simulink model "PX4MultiCopterPerceptionAndControl"  (R2026b)
settings: Solver=ode3  StopTime=inf
PreLoadFcn:
  | InitVars;
undefined symbols (not defined in the file): contact, control, dragCoeffMov, ft, g, gray, m, mass, NoOfRotors, NoOfRotorsSimulation, rotorDir, rotorPositions, rotorThrustMax, rotorTimeConst, rotorTorqueMax, s, SampleTime, Sim3dSensor, Sim3dVisualisationSampleTime, windVel
libraries: aerolibconvert2 x4, sim3dlib x4, slpidlib x4, shared6dof x1, visiongeotforms x1, sharedtransform x1, uavutilslib x1
settings Model: Creator=The MathWorks, Inc.  LastModifiedBy=Hirthick
settings OptimizationCC: DefaultParameterBehavior=Inlined  DifferentSizesBufferReuse=on  EfficientTunableParamExpr=on  EnhancedBackFolding=on  MaxStackSize=64  OptimizationCustomize=off  OptimizeBlockOrder=speed  PassReuseOutputArgsAs=Individual arguments  RemoveInternalMemoryZeroInit=on  RemoveRootLevelIOMemoryZeroInit=on
settings DebuggingCC: ArithmeticOperatorsInVariantConditions=warning  MergeDetectMultiDrivingBlocksExec=none  ParameterPrecisionLossMsg=none  ParameterTunabilityLossMsg=error
settings HardwareCC: ProdHWDeviceType=ARM Compatible->ARM Cortex  ProdLargestAtomicFloat=Double  ProdLargestAtomicInteger=Long
settings ModelReferenceCC: PropagateSignalLabelsOutOfModel=off
settings SFSimCC: MATLABDynamicMemAlloc=off
settings RTWCC: Description=Embedded Coder  SystemTargetFile=ert.tlc  TemplateMakefile=ert_default_tmf  Toolchain=GNU Tools for PX4 Autopilots
settings CodeAppCC: ForceParamTrailComments=on  IgnoreCustomStorageClasses=off  InsertBlockDesc=on  OperatorAnnotations=on  SFDataObjDesc=on  SimulinkDataObjDesc=on
settings ERTTargetCC: ExtModeIntrfLevel=Level2 - Open  ExtModeMexFile=ext_xcp  ExtModeStaticAlloc=on  SupportNonFinite=off  SupportVariableSizeSignals=on
settings ConfigComp: DVDefectChecker=on  DVDetectOutOfBounds=on  DVHarnessSource=Signal Editor  DVModelReferenceHarness=on  DVTestSuiteOptimization=Auto
settings SimscapeCC: SimscapeLogType=all  SimscapeNominalValues="[{\"value\":\"1\",\"unit\":\"A\"},{\"value\":\"1\",\"unit\":\"bar\"},{\"value\":\"1\",\"unit\":\"cm^2\"},{\"value\":\"1\",\"unit\":\"cm^3/s\"},{\"value\":\"1\",\"unit\":\"kJ/kg\"},{\"value\":\"1\",\"unit\":\"kW\"},{\"value\":\"1\",\"unit\":\"l\"},{\"value\":\"1\",\"unit\":\"N\"},{\"value\":\"1\",\"unit\":\"N*m\"},{\"value\":\"1\",\"unit\":\"V\"},{\"value\":\"0.001\",\"unit\":\"Wb\"}]"  SimscapeUseEnergyAccounting=off

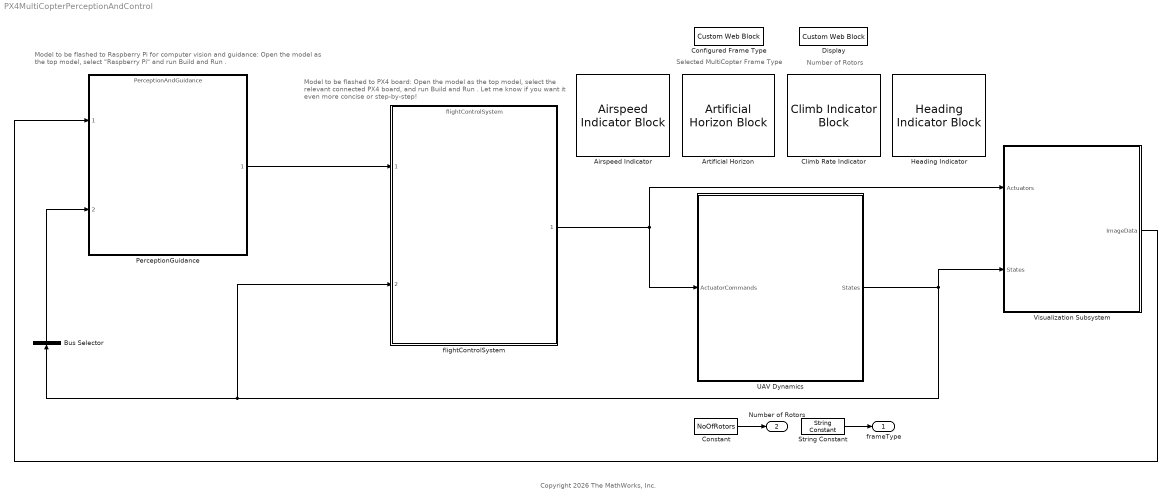
== system PX4MultiCopterPerceptionAndControl ==
  note: Selected MultiCopter Frame Type
  note: Number of Rotors
  note: Model to be flashed to Raspberry Pi for computer vision and guidance:
      | Open the model as the top model, select "Raspberry Pi" and run Build and Run .
  note: Model to be flashed to PX4 board:
      | Open the model as the top model, select the relevant connected PX4 board, and run Build and Run .
      | Let me know if you want it even more concise or step-by-step!
  note: Copyright 2026 The MathWorks, Inc.
  Airspeed Indicator : AirspeedIndicatorBlock  LabelPosition=Hide
  Artificial Horizon : ArtificialHorizonBlock  LabelPosition=Hide
  Bus Selector : BusSelector  OutputSignals=X,Y,Z,yaw  OutputAsBus=on
  Climb Rate Indicator : ClimbIndicatorBlock  LabelPosition=Hide
  "Configured Frame Type " : CustomWebBlock  LabelPosition=Hide  ShowInitialText=on  Configuration="{\"components\":[{\"name\":\"DisplayComponent\",\"settings\":{\"alignment\":\"center\",\"bold\":false,\"font\":\"Ubuntu\",\"fontColor\":[255,255,200],\"fontSize\":\"14\",\"format\":\"shortEng\",\"formatString\":\"%d\",\"gridColor\":[252,252,197],\"italic\":false,\"position\":[0,0,1,1],\"showGrid\":true,\"underline\":false}},{\"name\":\"BackgroundImageComponent\",\"settings\":{\"image\":{\"size\":[300,80],\"src\":\"data:image\\/svg+xml;base64,PHN2ZyBpZD0iZnJhbWUiIHhtbG5zPSJodHRwOi8vd3d3LnczLm9yZy8yMDAwL3N2ZyIgeG1sbnM6eGxpbms9Imh0dHA6Ly93d3cudzMub3JnLzE5OTkveGxpbmsiIHZpZXdCb3g9IjAgMCAzODAgMTAxIj48ZGVmcz48c3R5bGU+LmNscy0xe2ZpbGw6IzAwMmI0Mjt9LmNscy0ye2ZpbGw6IzQyNzA4Mjt9LmNscy0ze2ZpbGw6dXJsKCNyYWRpYWwtZ3JhZGllbnQpO308L3N0eWxlPjxyYWRpYWxHcmFkaWVudCBpZD0icmFkaWFsLWdyYWRpZW50IiBjeD0iMTkwIiBjeT0iNTAuNSIgcj0iMjY5LjIxIiBncmFkaWVudFVuaXRzPSJ1c2VyU3BhY2VPblVzZSI+PHN0b3Agb2Zmc2V0PSIwLjAxIiBzdG9wLWNvbG9yPSIjM2U0ZjU4Ii8+PHN0b3Agb2Zmc2V0PSIwLjA2IiBzdG9wLWNvbG9yPSIjNDQ1NzYxIi8+PHN0b3Agb2Zmc2V0PSIwLjE1IiBzdG9wLWNvbG9yPSIjNTU2YTc2Ii8+PHN0b3Agb2Zmc2V0PSIwLjI1IiBzdG9wLWNvbG9yPSIjNmQ4ODk1Ii8+PHN0b3Agb2Zmc2V0PSIwLjM4IiBzdG9wLWNvbG9yPSIjOGZiMmMzIi8+PHN0b3Agb2Zmc2V0PSIwLjUyIiBzdG9wLWNvbG9yPSIjYjZlNGZhIi8+PHN0b3Agb2Zmc2V0PSIxIiBzdG9wLWNvbG9yPSIjMTU0NjU3Ii8+PC9yYWRpYWxHcmFkaWVudD48L2RlZnM+PGcgaWQ9IkxheWVyXzIiIGRhdGEtbmFtZT0iTGF5ZXIgMiI+PGcgaWQ9IkxheWVyXzEtMiIgZGF0YS1uYW1lPSJMYXllciAxLTIiPjxyZWN0IGlkPSJyZWN0MTAzNiIgY2xhc3M9ImNscy0xIiB4PSIxMSIgeT0iMTEiIHdpZHRoPSIzNTgiIGhlaWdodD0iNzkiLz48cGF0aCBpZD0icGF0aDEwMzgiIGNsYXNzPSJjbHMtMiIgZD0iTTgsOFY5M0gzNzJWOFpNMzY5LDkwSDExVjExSDM2OVoiLz48cGF0aCBpZD0icGF0aDEwNDAiIGNsYXNzPSJjbHMtMyIgZD0iTTAsMFYxMDFIMzgwVjBaTTM3Miw5M0g4VjhIMzcyWiIvPjwvZz48L2c+PC9zdmc+\",\"srcOrientation\":\"Right\"},\"position\":[0,0,1,1],\"scaleMode\":\"0\"}},{\"name\":\"ForegroundImageComponent\",\"settings\":{\"angle\":0,\"image\":{\"size\":[0,0],\"src\":\"default\"},\"isForeground\":1,\"position\":[0,0,1,1],\"scaleMode\":\"0\"}}],\"derived\":{\"blockParameters\":{\"alignment\":\"center\",\"fixedAspectRatio\":\"on\",\"format\":\"shortEng\",\"formatString\":\"%d\",\"gridColor\":[252,252,197],\"showGrid\":true}},\"settings\":{\"BindingType\":\"signal\",\"aspectRatio\":1.032258064516129,\"backgroundColor\":[0,0,0,\"1\"],\"backgroundOffset\":0.14,\"backgroundOpacity\":1,\"fixedAspectRatio\":\"on\",\"showBackgroundColor\":false,\"value\":0,\"version\":\"R2026b\"},\"type\":\"Display\"}"  CustomBackgroundColor="{\"color\":[0.8509803921568627,0.8509803921568627,0.8509803921568627],\"show\":false}"
  Constant : Constant  Value=NoOfRotors  SampleTime=-1
  Display : CustomWebBlock  LabelPosition=Hide  ShowInitialText=on  Configuration="{\"components\":[{\"name\":\"DisplayComponent\",\"settings\":{\"alignment\":\"center\",\"bold\":false,\"font\":\"DSEG7 Classic\",\"fontColor\":[255,255,200],\"fontSize\":\"14\",\"format\":\"short\",\"formatString\":\"%d\",\"gridColor\":[252,252,197],\"italic\":false,\"position\":[0,0,1,1],\"showGrid\":true,\"underline\":false}},{\"name\":\"BackgroundImageComponent\",\"settings\":{\"image\":{\"size\":[300,80],\"src\":\"data:image\\/svg+xml;base64,PHN2ZyBpZD0iZnJhbWUiIHhtbG5zPSJodHRwOi8vd3d3LnczLm9yZy8yMDAwL3N2ZyIgeG1sbnM6eGxpbms9Imh0dHA6Ly93d3cudzMub3JnLzE5OTkveGxpbmsiIHZpZXdCb3g9IjAgMCAzODAgMTAxIj48ZGVmcz48c3R5bGU+LmNscy0xe2ZpbGw6IzAwMmI0Mjt9LmNscy0ye2ZpbGw6IzQyNzA4Mjt9LmNscy0ze2ZpbGw6dXJsKCNyYWRpYWwtZ3JhZGllbnQpO308L3N0eWxlPjxyYWRpYWxHcmFkaWVudCBpZD0icmFkaWFsLWdyYWRpZW50IiBjeD0iMTkwIiBjeT0iNTAuNSIgcj0iMjY5LjIxIiBncmFkaWVudFVuaXRzPSJ1c2VyU3BhY2VPblVzZSI+PHN0b3Agb2Zmc2V0PSIwLjAxIiBzdG9wLWNvbG9yPSIjM2U0ZjU4Ii8+PHN0b3Agb2Zmc2V0PSIwLjA2IiBzdG9wLWNvbG9yPSIjNDQ1NzYxIi8+PHN0b3Agb2Zmc2V0PSIwLjE1IiBzdG9wLWNvbG9yPSIjNTU2YTc2Ii8+PHN0b3Agb2Zmc2V0PSIwLjI1IiBzdG9wLWNvbG9yPSIjNmQ4ODk1Ii8+PHN0b3Agb2Zmc2V0PSIwLjM4IiBzdG9wLWNvbG9yPSIjOGZiMmMzIi8+PHN0b3Agb2Zmc2V0PSIwLjUyIiBzdG9wLWNvbG9yPSIjYjZlNGZhIi8+PHN0b3Agb2Zmc2V0PSIxIiBzdG9wLWNvbG9yPSIjMTU0NjU3Ii8+PC9yYWRpYWxHcmFkaWVudD48L2RlZnM+PGcgaWQ9IkxheWVyXzIiIGRhdGEtbmFtZT0iTGF5ZXIgMiI+PGcgaWQ9IkxheWVyXzEtMiIgZGF0YS1uYW1lPSJMYXllciAxLTIiPjxyZWN0IGlkPSJyZWN0MTAzNiIgY2xhc3M9ImNscy0xIiB4PSIxMSIgeT0iMTEiIHdpZHRoPSIzNTgiIGhlaWdodD0iNzkiLz48cGF0aCBpZD0icGF0aDEwMzgiIGNsYXNzPSJjbHMtMiIgZD0iTTgsOFY5M0gzNzJWOFpNMzY5LDkwSDExVjExSDM2OVoiLz48cGF0aCBpZD0icGF0aDEwNDAiIGNsYXNzPSJjbHMtMyIgZD0iTTAsMFYxMDFIMzgwVjBaTTM3Miw5M0g4VjhIMzcyWiIvPjwvZz48L2c+PC9zdmc+\",\"srcOrientation\":\"Right\"},\"position\":[0,0,1,1],\"scaleMode\":\"0\"}},{\"name\":\"ForegroundImageComponent\",\"settings\":{\"angle\":0,\"image\":{\"size\":[0,0],\"src\":\"default\"},\"isForeground\":1,\"position\":[0,0,1,1],\"scaleMode\":\"0\"}}],\"derived\":{\"blockParameters\":{\"alignment\":\"center\",\"fixedAspectRatio\":\"on\",\"format\":\"short\",\"formatString\":\"%d\",\"gridColor\":[252,252,197],\"showGrid\":true}},\"settings\":{\"BindingType\":\"signal\",\"aspectRatio\":1.032258064516129,\"backgroundColor\":[0,0,0,\"1\"],\"backgroundOffset\":0.14,\"backgroundOpacity\":1,\"fixedAspectRatio\":\"on\",\"showBackgroundColor\":false,\"value\":0,\"version\":\"R2026b\"},\"type\":\"Display\"}"
  Heading Indicator : HeadingIndicatorBlock  LabelPosition=Hide
  PerceptionGuidance : ModelReference  ModelNameDialog=PerceptionAndGuidance.slx  SimulationMode=Normal  ModelReferenceVersion=7.101
  String Constant : StringConstant  String=frameType
  UAV Dynamics : Subsystem
  Visualization Subsystem : Subsystem
  flightControlSystem : ModelReference  ModelNameDialog=flightControlSystem.slx  SimulationMode=Normal  ModelReferenceVersion=11.62
  frameType : Outport
  Number of Rotors : Outport  Port=2
  wires:
  flightControlSystem/1 -> Visualization Subsystem/1(Actuators), UAV Dynamics/1(ActuatorCommands)
  String Constant/1 -> frameType/1
  Constant/1 -> Number of Rotors/1
  PerceptionGuidance/1 -> flightControlSystem/1
  UAV Dynamics/1(States) -> Bus Selector/1, flightControlSystem/2, Visualization Subsystem/2(States)
  Bus Selector/1 -> PerceptionGuidance/2
  Visualization Subsystem/1(ImageData) -> PerceptionGuidance/1

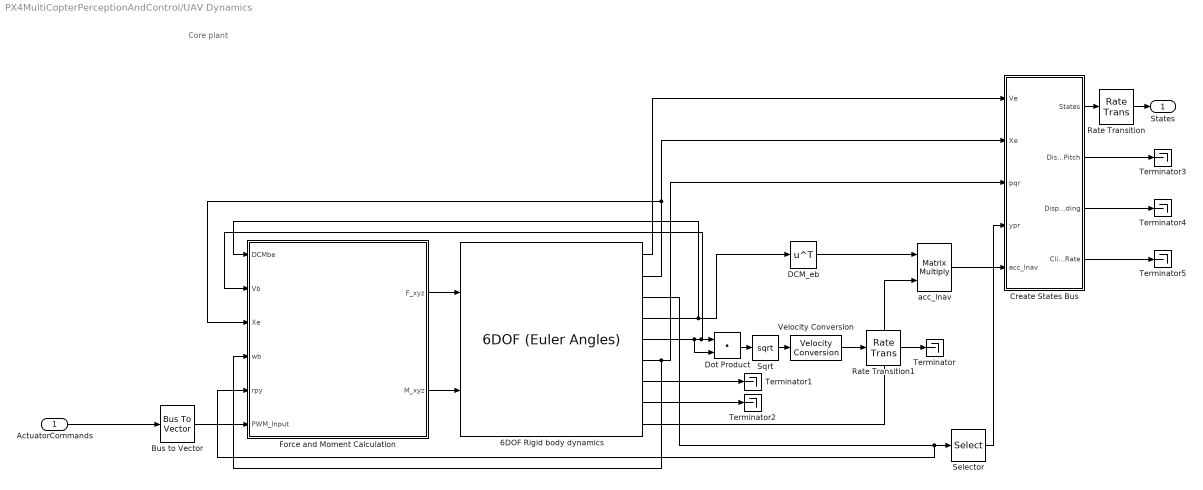
== system PX4MultiCopterPerceptionAndControl/UAV Dynamics ==
  note: Core plant
  ActuatorCommands : Inport  OutDataTypeStr=Bus: setPWMInput
  "6DOF Rigid body dynamics " : shared6dof/6DOF (Euler Angles)  units=Metric (MKS)  mtype=Fixed  rep=Euler Angles  xme_0=init.posNED  Vm_0=init.vb  eul_0=[0,0,0]  pm_0=init.angRates  mass_0=mass  mass_e=0.5  mass_f=2.0  inertia=inertia  inertia_e=eye(3)  inertia_f=2*eye(3)  k_quat=Vehicle.SixDOF.quatGain  vre_flag=on  abi_flag=on  aMode=aMode  xme_statename=''  Vm_statename=''  eul_statename=''  quat_statename=''  pm_statename=''  mass_statename=''
  Bus to Vector : BusToVector
  Create States Bus : Subsystem
  DCM_eb : Math  Operator=transpose
  Dot Product : DotProduct  OutDataTypeStr=Inherit: Inherit via internal rule
  Force and Moment Calculation : Subsystem
  Rate Transition : RateTransition  OutPortSampleTime=SampleTime
  Rate Transition1 : RateTransition
  Selector : Selector  InputPortWidth=3  IndexOptions=Index vector (dialog)  Indices=[3 2 1]  OutputSizes=1
  Sqrt : Sqrt
  Terminator{,1..5} (6 alike) : Terminator
  Velocity Conversion : aerolibconvert2/Velocity Conversion  IU=m/s  OU=kts
  acc_lnav : Product  Multiplication=Matrix(*)
  States : Outport  OutDataTypeStr=Bus: UAVStatesBus
  wires:
  "6DOF Rigid body dynamics "/3 -> Force and Moment Calculation/5(rpy), Selector/1
  "6DOF Rigid body dynamics "/8 -> Terminator2/1
  "6DOF Rigid body dynamics "/4 -> Force and Moment Calculation/1(DCMbe), DCM_eb/1
  "6DOF Rigid body dynamics "/2 -> Create States Bus/2(Xe), Force and Moment Calculation/3(Xe)
  "6DOF Rigid body dynamics "/1 -> Create States Bus/1(Ve)
  acc_lnav/1 -> Create States Bus/5(acc_lnav)
  Bus to Vector/1 -> Force and Moment Calculation/6(PWM_Input)
  "6DOF Rigid body dynamics "/7 -> Terminator1/1
  Selector/1 -> Create States Bus/4(ypr)
  Force and Moment Calculation/1(F_xyz) -> "6DOF Rigid body dynamics "/1
  DCM_eb/1 -> acc_lnav/1
  "6DOF Rigid body dynamics "/5 -> Dot Product/1, Force and Moment Calculation/2(Vb), Dot Product/2
  "6DOF Rigid body dynamics "/6 -> Force and Moment Calculation/4(wb), Create States Bus/3(pqr)
  ActuatorCommands/1 -> Bus to Vector/1
  "6DOF Rigid body dynamics "/9 -> acc_lnav/2
  Force and Moment Calculation/2(M_xyz) -> "6DOF Rigid body dynamics "/2
  Create States Bus/1(States) -> Rate Transition/1
  Rate Transition/1 -> States/1
  Create States Bus/2(DisplayRollPitch) -> Terminator3/1
  Create States Bus/3(DisplayHeading) -> Terminator4/1
  Velocity Conversion/1 -> Rate Transition1/1
  Sqrt/1 -> Velocity Conversion/1
  Dot Product/1 -> Sqrt/1
  Create States Bus/4(ClimbRate) -> Terminator5/1
  Rate Transition1/1 -> Terminator/1

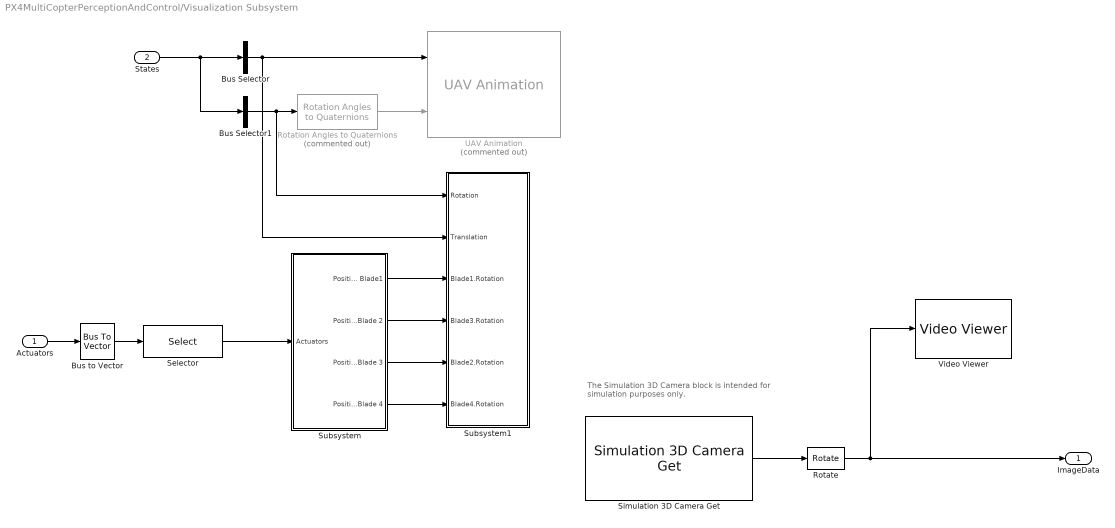
== system PX4MultiCopterPerceptionAndControl/Visualization Subsystem ==
  note: The Simulation 3D Camera block is intended for simulation purposes only.
  Actuators : Inport
  States : Inport  Port=2
  Bus Selector : BusSelector  OutputSignals=X,Y,Z  OutputAsBus=on
  Bus Selector1 : BusSelector  OutputSignals=yaw,pitch,roll  OutputAsBus=on
  Bus to Vector : BusToVector
  Rotate : visiongeotforms/Rotate  outSizeR=Expanded to fit rotated input image  src_angle=Specify via dialog  unit_angle=Degrees  angle=pi/2  maxAngle=pi  dispImage=Top-left corner  method=Table lookup  fillVal=0  interpMethod=Bilinear  roundingMode=Nearest  overflowMode=on  prodOutputMode=Binary point scaling  prodOutputWordLength=32  prodOutputFracLength=10
  Rotation Angles to Quaternions : sharedtransform/Rotation Angles to Quaternions  Commented=on  rotationOrder=ZYX  aMode=aMode
  Selector : Selector  InputPortWidth=8  IndexOptions=Index vector (dialog)  Indices=1:NoOfRotorsSimulation  OutputSizes=1
  Simulation 3D Camera Get : sim3dlib/Simulation 3D Camera Get  Priority=1  sensorTag=Sim3dSensor�  sensorId=1  sensorName=Sim3dSensor�  vehTagList={'Custom ...';'Quadcopter';'Scene Origin';'Sim3dActor1'}  vehTag=Quadcopter  CoordinateSystem=VRML  mountLoc=Origin  offsetFlag=on  tmountOffset=[0, -0.1, 0]  rmountOffset=[0, deg2rad(-90), deg2rad(90)]  HorizontalResolution=120  VerticalResolution=160  HorizontalFOV=38  SampleTime=0.2  mountPoint=[0 -0.1 0]  mountOrientation=[0 1.5707963267949 -1.5707963267949]  aMode=5  ID=1
      settings: LibrarySourceBlock=sl3dlib/Simulation 3D/Utilities/Simulation 3D Camera Get
  Subsystem : Subsystem
  Subsystem1 : Subsystem
  UAV Animation : uavutilslib/UAV Animation  Commented=on  NumUAV=1  DynamicUAVConfig=off  UAVType=Multirotor  UAVSize=1  UAVColor=[1 0 0]  UAVTrajectoryAlpha=1  AlwaysShowAnimation=on  AxisLimits=[-Inf Inf;-Inf Inf;-Inf Inf]  TrajectoryBufferSize=100000  InertialZDirection=Down  RotationFormat=Quaternion  DrawMarkers=off  SampleTime=Sim3dVisualisationSampleTime
  Video Viewer : VideoViewer  colormapValue=gray(256)  FigPos=[261 843.666666666667 419 306]
  ImageData : Outport
  wires:
  States/1 -> Bus Selector1/1, Bus Selector/1
  Subsystem/2(Position Blade 2) -> Subsystem1/4(Blade3.Rotation)
  Subsystem/4(Position Blade 4) -> Subsystem1/6(Blade4.Rotation)
  Subsystem/3(Position Blade 3) -> Subsystem1/5(Blade2.Rotation)
  Subsystem/1(Position Blade1) -> Subsystem1/3(Blade1.Rotation)
  Rotation Angles to Quaternions/1 -> UAV Animation/2
  Actuators/1 -> Bus to Vector/1
  Bus Selector1/1 -> Subsystem1/1(Rotation), Rotation Angles to Quaternions/1
  Bus Selector/1 -> Subsystem1/2(Translation), UAV Animation/1
  Selector/1 -> Subsystem/1(Actuators)
  Bus to Vector/1 -> Selector/1
  Simulation 3D Camera Get/1 -> Rotate/1
  Rotate/1 -> ImageData/1, Video Viewer/1

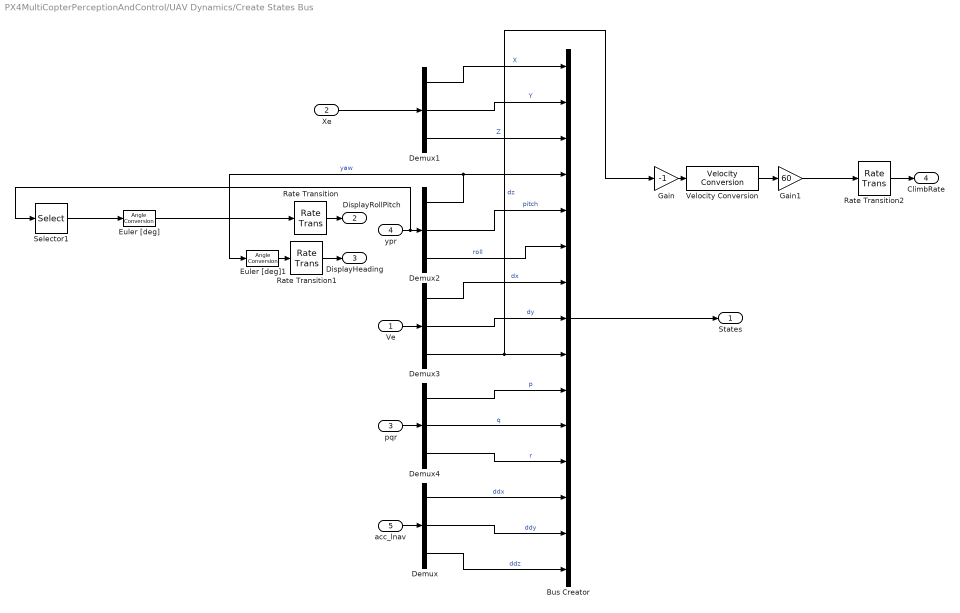
== system PX4MultiCopterPerceptionAndControl/UAV Dynamics/Create States Bus ==
  Ve : Inport
  Xe : Inport  Port=2
  pqr : Inport  Port=3
  ypr : Inport  Port=4
  acc_lnav : Inport  Port=5
  Bus Creator : BusCreator  Inputs=15
  Demux{,1..4} (5 alike) : Demux  Outputs=3
  Euler [deg] : aerolibconvert2/Angle Conversion  IU=rad  OU=deg
  Euler [deg]1 : aerolibconvert2/Angle Conversion  IU=rad  OU=deg
  Gain : Gain  Gain=-1
  Gain1 : Gain  Gain=60
  Rate Transition : RateTransition
  Rate Transition1 : RateTransition
  Rate Transition2 : RateTransition
  Selector1 : Selector  InputPortWidth=3  IndexOptions=Index vector (dialog)  Indices=[3 2]  OutputSizes=1
  Velocity Conversion : aerolibconvert2/Velocity Conversion  IU=m/s  OU=ft/s
  States : Outport
  DisplayRollPitch : Outport  Port=2
  DisplayHeading : Outport  Port=3
  ClimbRate : Outport  Port=4
  wires:
  Demux/1 -> Bus Creator/13  "ddx"
  Xe/1 -> Demux1/1
  acc_lnav/1 -> Demux/1
  Ve/1 -> Demux3/1
  pqr/1 -> Demux4/1
  Demux1/3 -> Bus Creator/3  "Z"
  Demux1/1 -> Bus Creator/1  "X"
  Demux1/2 -> Bus Creator/2  "Y"
  Demux2/1 -> Euler [deg]1/1, Bus Creator/4  "yaw"
  Demux2/2 -> Bus Creator/5  "pitch"
  Demux2/3 -> Bus Creator/6  "roll"
  Demux3/1 -> Bus Creator/7  "dx"
  Demux4/3 -> Bus Creator/12  "r"
  Demux3/2 -> Bus Creator/8  "dy"
  Demux3/3 -> Gain/1, Bus Creator/9  "dz"
  Demux4/1 -> Bus Creator/10  "p"
  Demux4/2 -> Bus Creator/11  "q"
  Demux/2 -> Bus Creator/14  "ddy"
  Demux/3 -> Bus Creator/15  "ddz"
  Bus Creator/1 -> States/1
  ypr/1 -> Selector1/1, Demux2/1
  Selector1/1 -> Euler [deg]/1
  Euler [deg]/1 -> Rate Transition/1
  Gain/1 -> Velocity Conversion/1
  Velocity Conversion/1 -> Gain1/1
  Gain1/1 -> Rate Transition2/1
  Euler [deg]1/1 -> Rate Transition1/1
  Rate Transition/1 -> DisplayRollPitch/1
  Rate Transition1/1 -> DisplayHeading/1
  Rate Transition2/1 -> ClimbRate/1

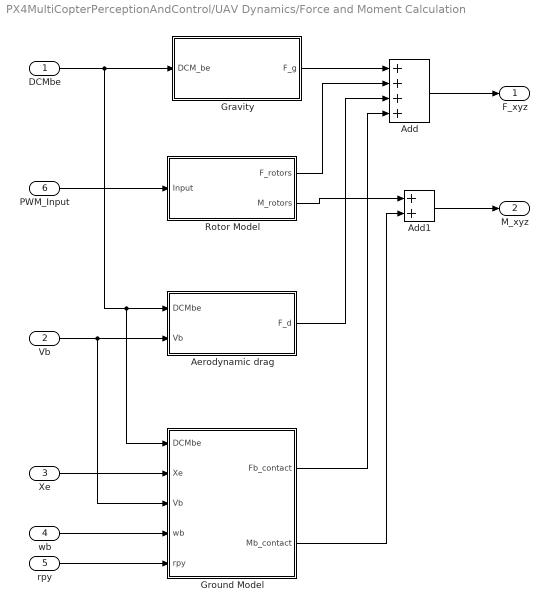
== system PX4MultiCopterPerceptionAndControl/UAV Dynamics/Force and Moment Calculation ==
  DCMbe : Inport
  Vb : Inport  Port=2
  Xe : Inport  Port=3
  wb : Inport  Port=4
  rpy : Inport  Port=5
  PWM_Input : Inport  Port=6
  Add : Sum  Inputs=++++
  Add1 : Sum
  Aerodynamic drag : Subsystem
  Gravity : Subsystem
  Ground Model : Subsystem
  Rotor Model : Subsystem
  F_xyz : Outport
  M_xyz : Outport  Port=2
  wires:
  PWM_Input/1 -> Rotor Model/1(Input)
  Gravity/1(F_g) -> Add/1
  Rotor Model/1(F_rotors) -> Add/2
  Aerodynamic drag/1(F_d) -> Add/3
  Ground Model/1(Fb_contact) -> Add/4
  Vb/1 -> Ground Model/3(Vb), Aerodynamic drag/2(Vb)
  DCMbe/1 -> Ground Model/1(DCMbe), Aerodynamic drag/1(DCMbe), Gravity/1(DCM_be)
  Xe/1 -> Ground Model/2(Xe)
  wb/1 -> Ground Model/4(wb)
  rpy/1 -> Ground Model/5(rpy)
  Rotor Model/2(M_rotors) -> Add1/1
  Ground Model/2(Mb_contact) -> Add1/2
  Add1/1 -> M_xyz/1
  Add/1 -> F_xyz/1

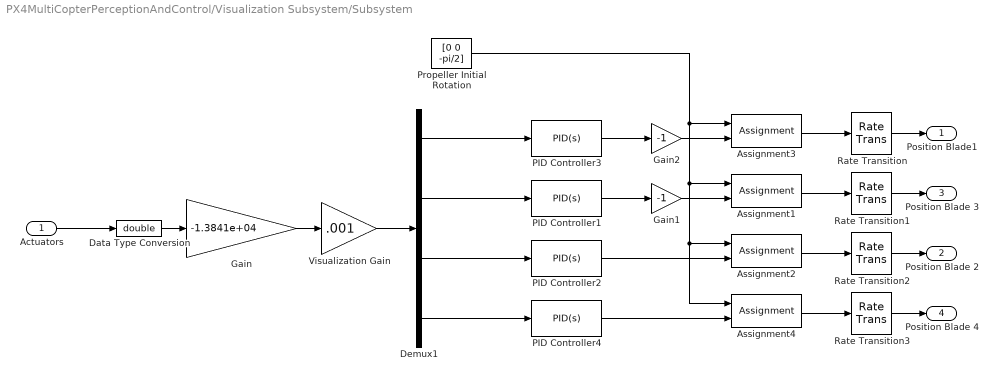
== system PX4MultiCopterPerceptionAndControl/Visualization Subsystem/Subsystem ==
  Actuators : Inport
  Assignment{1..4} (4 alike) : Assignment  DiagnosticForDimensions=Warning  IndexOptions=Index vector (dialog)  Indices=3  OutputSizes=1
  Data Type Conversion : DataTypeConversion  OutDataTypeStr=double  SaturateOnIntegerOverflow=off  RndMeth=Floor
  Demux1 : Demux
  Gain : Gain  Gain=-1.3841e+04
  Gain1 : Gain  Gain=-1
  Gain2 : Gain  Gain=-1
  PID Controller{1..4} (4 alike) : slpidlib/PID Controller  Controller=PID  Form=Parallel  TimeDomain=Continuous-time  UseExternalTs=off  SampleTime=-1  IntegratorMethod=Forward Euler  FilterMethod=Forward Euler  ControllerParametersSource=internal  P=1  I=1.5  UseKiTs=off  D=0  UseExternalDerivativeSource=off  N=100  UseFilter=on  TunerSelectOption=Transfer Function Based (PID Tuner App)  InitialConditionSource=internal  InitialConditionForIntegrator=0  InitialConditionForFilter=0  DifferentiatorICPrevScaledInput=0  ExternalReset=none  TrackingMode=off  Kt=1  LimitOutput=off  SatLimitsSource=internal  UpperSaturationLimit=inf  LowerSaturationLimit=-inf  LinearizeAsGain=on  AntiWindupMode=none  Kb=1  LimitIntegrator=off  UpperIntegratorSaturationLimit=inf  LowerIntegratorSaturationLimit=-inf  POutMin=[]  POutMax=[]  IOutMin=[]  IOutMax=[]  DOutMin=[]  DOutMax=[]  NOutMin=[]  NOutMax=[]  SumOutMin=[]  SumOutMax=[]  SaturationOutMin=[]  SaturationOutMax=[]  PParamMin=[]  PParamMax=[]  IParamMin=[]  IParamMax=[]  DParamMin=[]  DParamMax=[]  NParamMin=[]  NParamMax=[]  KbParamMin=[]  KbParamMax=[]  KtParamMin=[]  KtParamMax=[]  KbOutMin=[]  KbOutMax=[]  KtOutMin=[]  KtOutMax=[]  IntegratorOutMin=[]  IntegratorOutMax=[]  FilterOutMin=[]  FilterOutMax=[]  SumI1OutMin=[]  SumI1OutMax=[]  SumI2OutMin=[]  SumI2OutMax=[]  SumI3OutMin=[]  SumI3OutMax=[]  SumI4OutMin=[]  SumI4OutMax=[]  SumDOutMin=[]  SumDOutMax=[]  DifferentiatorOutMin=[]  DifferentiatorOutMax=[]  FilterDiffOutCoefMin=[]  FilterDiffOutCoefMax=[]  ReciprocalOutMin=[]  ReciprocalOutMax=[]  SumDenOutMin=[]  SumDenOutMax=[]  SumNumOutMin=[]  SumNumOutMax=[]  DivideOutMin=[]  DivideOutMax=[]  UdiffTsProdOutMin=[]  UdiffTsProdOutMax=[]  NTsProdOutMin=[]  NTsProdOutMax=[]  UintegralTsProdOutMin=[]  UintegralTsProdOutMax=[]  UngainTsProdOutMin=[]  UngainTsProdOutMax=[]  ClampingZeroOutDataTypeStr=Inherit: Inherit via back propagation  ClampingZeroOutMin=[]  ClampingZeroOutMax=[]  FilterDenConstantOutDataTypeStr=Inherit: Inherit via back propagation  FilterDenConstantOutMin=[]  FilterDenConstantOutMax=[]  PCopyOutDataTypeStr=Inherit: Inherit via back propagation  PCopyOutMin=[]  PCopyOutMax=[]  NCopyOutDataTypeStr=Inherit: Inherit via back propagation  NCopyOutMin=[]  NCopyOutMax=[]  IntegratorContinuousStateAttributes=''  IntegratorStateMustResolveToSignalObject=off  IntegratorRTWStateStorageClass=Auto  FilterContinuousStateAttributes=''  FilterStateMustResolveToSignalObject=off  FilterRTWStateStorageClass=Auto  ParallelPVariant=InternalParameters  IdealPVariant=Disabled  IVariant=InternalParameters  DVariant=InternalParameters  IntegratorVariant=Continuous  SatVariant=Disabled  AWVariant=Passthrough  PCopyVariant=Disabled  TRVariant=Disabled  FdbkBlocksVariant=Forward  IdealPFdbkVariant=Disabled  SatFdbkVariant=Disabled  DerivativeFilterVariant=ContFilter  NVariant=InternalParameters  NCopyVariant=Disabled  FilterICVariant=InternalICsFilter  IntegratorICVariant=InternalICs  ExternalResetVariant=Disabled  TRSumVariant=Passthrough  SumFdbkVariant=Disabled  SumVariant=Sum_PID  TsampFilterVariant=InternalTs  TsampNgainVariant=Passthrough  TsampIntegralVariant=Disabled_SignalSpec  ExternalSaturationOutDataTypeStr=Inherit: Same as second input  DerivativeSourceVariant=ErrorSignal  PreIntVariant=InternalPreInt
  Propeller Initial Rotation : Constant  Value=[0 0 -pi/2]  VectorParams1D=off  SampleTime=Sim3dVisualisationSampleTime
  Rate Transition{,1..3} (4 alike) : RateTransition
  Visualization Gain : Gain  Gain=.001
  Position Blade1 : Outport  VectorParamsAs1DForOutWhenUnconnected=off
  Position Blade 2 : Outport  Port=2  VectorParamsAs1DForOutWhenUnconnected=off
  Position Blade 3 : Outport  Port=3  VectorParamsAs1DForOutWhenUnconnected=off
  Position Blade 4 : Outport  Port=4  VectorParamsAs1DForOutWhenUnconnected=off
  wires:
  Actuators/1 -> Data Type Conversion/1
  Demux1/3 -> PID Controller2/1
  Data Type Conversion/1 -> Gain/1
  Gain/1 -> Visualization Gain/1
  Visualization Gain/1 -> Demux1/1
  Demux1/1 -> PID Controller3/1
  Demux1/2 -> PID Controller1/1
  Demux1/4 -> PID Controller4/1
  Propeller Initial Rotation/1 -> Assignment2/1, Assignment4/1, Assignment1/1, Assignment3/1
  Assignment1/1 -> Rate Transition1/1
  Assignment3/1 -> Rate Transition/1
  Assignment2/1 -> Rate Transition2/1
  Assignment4/1 -> Rate Transition3/1
  PID Controller4/1 -> Assignment4/2
  PID Controller3/1 -> Gain2/1
  PID Controller1/1 -> Gain1/1
  PID Controller2/1 -> Assignment2/2
  Gain2/1 -> Assignment3/2
  Rate Transition/1 -> Position Blade1/1
  Rate Transition1/1 -> Position Blade 3/1
  Rate Transition2/1 -> Position Blade 2/1
  Rate Transition3/1 -> Position Blade 4/1
  Gain1/1 -> Assignment1/2

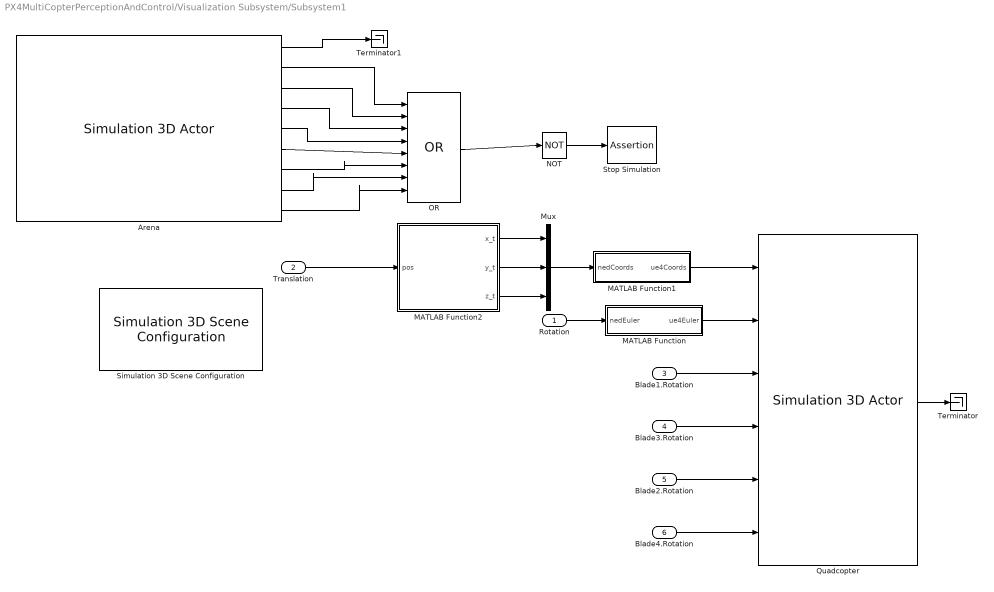
== system PX4MultiCopterPerceptionAndControl/Visualization Subsystem/Subsystem1 ==
  Rotation : Inport
  Translation : Inport  Port=2
  Blade1.Rotation : Inport  Port=3
  Blade3.Rotation : Inport  Port=4
  Blade2.Rotation : Inport  Port=5
  Blade4.Rotation : Inport  Port=6
  Arena : sim3dlib/Simulation 3D Actor  Priority=1  ActorName=Sim3dActor1  ParentName=Scene Origin  Operation=Create at setup  InitScriptText=|  SampleTime=Sim3dVisualisationSampleTime  Translation=single([0 0 0])  Rotation=single([0 0 0])  Scale=single([1 1 1])  EventsText=|  aMode=5  ActorTag=Sim3dActor1  ActorType=Sim3dActor  ID=1
      InitScriptText=|
      | % Reserved keywords:
      | % - Actor : handle to this actor object
      | % - World : handle to the world object
      | 
      | % Examples:
      | 
      | % Create a primitive geometry (optional)
      | % createShape(Actor, 'box', [1 1 1]);
      | 
      | % Initialize values (optional)
      | % Actor.Physics = true;
      | % Actor.Color = [1 0 0];
      EventsText=|
      | pillar1.BeginOverlapEvent
      | pillar2.BeginOverlapEvent
      | pillar3.BeginOverlapEvent
      | pillar4.BeginOverlapEvent
      | wall.BeginOverlapEvent   
      | wall_2.BeginOverlapEvent 
      | wall_3.BeginOverlapEvent 
      | wall_4.BeginOverlapEvent
  MATLAB Function : MATLAB Function  TreatAsAtomicUnit=on
  MATLAB Function1 : MATLAB Function  TreatAsAtomicUnit=on
  MATLAB Function2 : MATLAB Function  TreatAsAtomicUnit=on
  Mux : Mux  Inputs=3
  NOT : Logic  Operator=NOT  IconShape=distinctive  AllPortsSameDT=off  OutDataTypeStr=boolean
  OR : Logic  Operator=OR  Inputs=8  IconShape=distinctive  AllPortsSameDT=off  OutDataTypeStr=boolean
  Quadcopter : sim3dlib/Simulation 3D Actor  Priority=1  ActorName=Quadcopter  ParentName=Scene Origin  Operation=Create at setup  InitScriptText=|  SampleTime=Sim3dVisualisationSampleTime  Translation=single([0 0 0])  Rotation=single([0 0 -90])  Scale=single([1 1 1])  InputsText=|  aMode=5  ActorTag=Quadcopter  ActorType=Sim3dActor  ID=C
      InitScriptText=|
      | fileName = fullfile(fileparts(fileparts(get_param(bdroot,'FileName'))), 'support','Quadcopter.mat');
      | Actor.load(fileName);
      | Actor.Mobility=sim3d.utils.MobilityTypes.Movable;
      | World.Actors.QuadBody.Collisions = 0; % Disable Collisions
      | % propagate(World.Actors.QuadBody, 'OverlapEventEnabled',true);
      | % World.Actors.QuadBody.Translation = [-1.5 -1 0.05];
      InputsText=|
      | Quadcopter.Translation
      | Quadcopter.Rotation   
      | Prop_FR.Rotation      
      | Prop_FL.Rotation      
      | Prop_RL.Rotation      
      | Prop_RR.Rotation
  Simulation 3D Scene Configuration : sim3dlib/Simulation 3D Scene Configuration  Priority=0  EnableWindow=on  ViewerType=Default Viewer  ProjectFormat=Default Scenes  SceneDesc=US city block  ProjectName=D:\MATLAB\toolbox\shared\sim3d_projects\automotive_project_windows\UE\WindowsNoEditor\VehicleSimulation.exe  ScenePath=/Game/Maps/HwStrght  EnableOpenDRIVE=off  vehTagList={'Custom';'Quadcopter';'Scene Origin';'Sim3dActor1'}  vehTag=Quadcopter  AttachedCameraRelativeTranslation=[0 0 1]  FreeCameraDefaultInitialTranslation=[-6, 0, 2]  AttachedCameraRelativeRotation=[0 -90 0]  FreeCameraDefaultInitialRotation=[0, -15, 0]  ViewpointName=Custom  FreeCameraInitialTranslation=[2 2 6]  FreeCameraInitialRotation=[0 -90 0]  OpVisEn=off  Ts=Sim3dVisualisationSampleTime  EnableRemoteAccess=off  SimulationMode=CoSimulation  SimulateUsing=Interpreted execution  EnableAnimationRecording=off  OverrideDefaultRecording=off  AnimationRecordingFileName=sim3dAnimation.mat  AnimationRecordingInterval=[0 inf]  EnableWeather=off  SunAzimuth=90  SunAltitude=40.0  EnableGeospatialSun=off  Latitude=0  Longitude=0  Date=2023-01-01  Time=10:30:00  GeoTimeZone=-5.0  SunDaylightSaving=off  wind=1  clouds=10  EnableVolumetricClouds=off  CloudCoverage=0  CloudAltitude=6  fog=0  rain=0  RaindropsEffect=off  SnowDensity=0  EnableGeospatial=off  TilesetSource=Earth terrain  UseTrueOrigin=off  OriginHeight=200  OriginLatitude=40.744652  OriginLongitude=-73.988864  MapStyle=Aerial  AdditionalAssetIDs=[]  UseAdvancedSunSky=off  SolarTime=11  TimeZone=-5  Day=21  Month=9  Year=2022  UseDaylightSavingTime=on  DSTStartDay=10  DSTStartMonth=3  DSTEndDay=3  DSTEndMonth=11  DSTSwitchHour=2  sensorTag=MainCamera1  sensorId=1  sensorName=MainCamera1  mountLoc=Origin  offsetFlag=off  tmountOffset=[0, 0, 0]  rmountOffset=[0, 0, 0]  HorizontalResolution=1280  VerticalResolution=720  HorizontalFOV=60  mountPoint=[0 0 0]  mountOrientation=[0 0 0]  aMode=5  ID=1  GeoTrigger=Inactive  ViewNameList={'Custom'}  ViewTranslationList={'[2 2 6]'}  ViewRotationList={'[0 -90 0]'}
      settings: LibrarySourceBlock=sl3dlib/Simulation 3D/Environment/Simulation 3D Scene Configuration
  Stop Simulation : Assertion  AssertionFailFcn=error('The model has stopped as the drone hit the boundary.')
  Terminator : Terminator
  Terminator1 : Terminator
  wires:
  Arena/1 -> Terminator1/1
  MATLAB Function2/3(z_t) -> Mux/3
  Arena/2 -> OR/1
  Arena/3 -> OR/2
  Arena/4 -> OR/3
  Arena/5 -> OR/4
  OR/1 -> NOT/1
  MATLAB Function2/1(x_t) -> Mux/1
  MATLAB Function2/2(y_t) -> Mux/2
  NOT/1 -> Stop Simulation/1
  Rotation/1 -> MATLAB Function/1(nedEuler)
  MATLAB Function1/1(ue4Coords) -> Quadcopter/1
  Blade1.Rotation/1 -> Quadcopter/3
  Blade3.Rotation/1 -> Quadcopter/4
  Blade2.Rotation/1 -> Quadcopter/5
  Blade4.Rotation/1 -> Quadcopter/6
  Quadcopter/1 -> Terminator/1
  MATLAB Function/1(ue4Euler) -> Quadcopter/2
  Arena/6 -> OR/5
  Arena/7 -> OR/6
  Arena/8 -> OR/7
  Arena/9 -> OR/8
  Translation/1 -> MATLAB Function2/1(pos)
  Mux/1 -> MATLAB Function1/1(nedCoords)

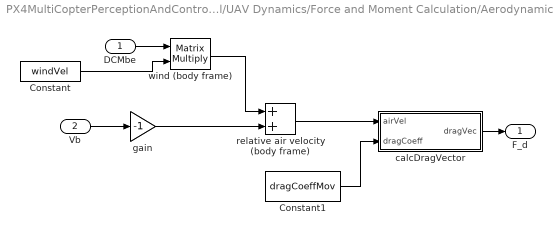
== system PX4MultiCopterPerceptionAndControl/UAV Dynamics/Force and Moment Calculation/Aerodynamic drag ==
  DCMbe : Inport
  Vb : Inport  Port=2
  Constant : Constant  Value=windVel
  Constant1 : Constant  Value=dragCoeffMov  SampleTime=-1
  calcDragVector : MATLAB Function  TreatAsAtomicUnit=on
  gain : Gain  Gain=-1
  relative air velocity (body frame) : Sum
  wind (body frame) : Product  Multiplication=Matrix(*)
  F_d : Outport
  wires:
  Vb/1 -> gain/1
  calcDragVector/1(dragVec) -> F_d/1
  relative air velocity (body frame)/1 -> calcDragVector/1(airVel)
  gain/1 -> relative air velocity (body frame)/2
  Constant1/1 -> calcDragVector/2(dragCoeff)
  DCMbe/1 -> wind (body frame)/1
  Constant/1 -> wind (body frame)/2
  wind (body frame)/1 -> relative air velocity (body frame)/1

== system PX4MultiCopterPerceptionAndControl/UAV Dynamics/Force and Moment Calculation/Gravity ==
  DCM_be : Inport
  Constant : Constant  Value=[0 0 g]'
  Gain : Gain  Gain=mass
  Matrix Multiply : Product  Multiplication=Matrix(*)
  F_g : Outport
  wires:
  Matrix Multiply/1 -> Gain/1
  Constant/1 -> Matrix Multiply/2
  DCM_be/1 -> Matrix Multiply/1
  Gain/1 -> F_g/1

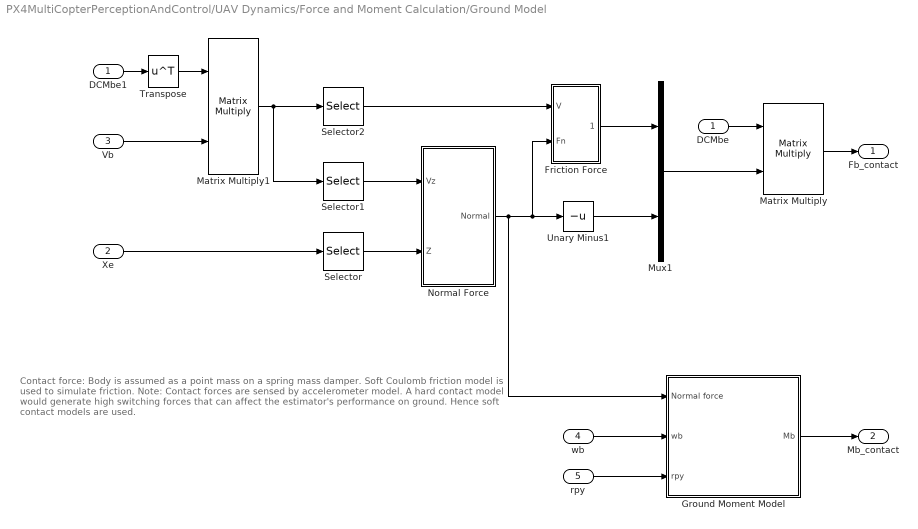
== system PX4MultiCopterPerceptionAndControl/UAV Dynamics/Force and Moment Calculation/Ground Model ==
  note: Contact force:
      | Body is assumed as a point mass on a spring mass damper. Soft Coulomb friction model is used to simulate friction.
      |
      | Note:
      | Contact forces are sensed by accelerometer model. A hard contact model would generate high switching forces that can affect the estimator's performance on ground. Hence soft contact models are used.
  DCMbe : Inport
  Xe : Inport  Port=2
  Vb : Inport  Port=3
  wb : Inport  Port=4
  rpy : Inport  Port=5
  DCMbe1 : InportShadow
  Friction Force : Subsystem
  Ground Moment Model : Subsystem
  Matrix Multiply : Product  Multiplication=Matrix(*)
  Matrix Multiply1 : Product  Multiplication=Matrix(*)
  Mux1 : Mux  Inputs=2
  Normal Force : Subsystem
  Selector : Selector  InputPortWidth=3  IndexOptions=Index vector (dialog)  Indices=[3]  OutputSizes=1
  Selector1 : Selector  InputPortWidth=3  IndexOptions=Index vector (dialog)  Indices=[3]  OutputSizes=1
  Selector2 : Selector  InputPortWidth=3  IndexOptions=Index vector (dialog)  Indices=[1,2]  OutputSizes=1
  Transpose : Math  Operator=transpose
  Unary Minus1 : UnaryMinus
  Fb_contact : Outport
  Mb_contact : Outport  Port=2
  wires:
  Xe/1 -> Selector/1
  Selector1/1 -> Normal Force/1(Vz)
  Selector/1 -> Normal Force/2(Z)
  DCMbe/1 -> Matrix Multiply/1
  Matrix Multiply/1 -> Fb_contact/1
  Normal Force/1(Normal) -> Ground Moment Model/1(Normal force), Unary Minus1/1, Friction Force/2(Fn)
  Mux1/1 -> Matrix Multiply/2
  Unary Minus1/1 -> Mux1/2
  Selector2/1 -> Friction Force/1(V)
  Friction Force/1(Friction) -> Mux1/1
  DCMbe1/1 -> Transpose/1
  Transpose/1 -> Matrix Multiply1/1
  Vb/1 -> Matrix Multiply1/2
  Matrix Multiply1/1 -> Selector1/1, Selector2/1
  Ground Moment Model/1(Mb) -> Mb_contact/1
  wb/1 -> Ground Moment Model/2(wb)
  rpy/1 -> Ground Moment Model/3(rpy)

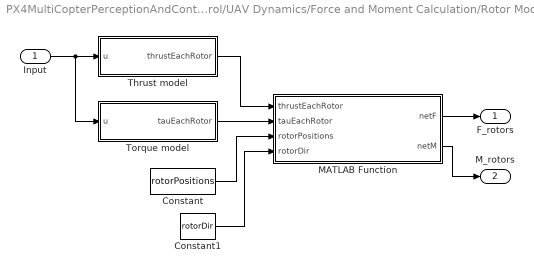
== system PX4MultiCopterPerceptionAndControl/UAV Dynamics/Force and Moment Calculation/Rotor Model ==
  Input : Inport
  Constant : Constant  Value=rotorPositions  SampleTime=-1
  Constant1 : Constant  Value=rotorDir  SampleTime=-1
  MATLAB Function : MATLAB Function  TreatAsAtomicUnit=on
  Thrust model : Subsystem
  Torque model : Subsystem
  F_rotors : Outport
  M_rotors : Outport  Port=2
  wires:
  MATLAB Function/1(netF) -> F_rotors/1
  Constant1/1 -> MATLAB Function/4(rotorDir)
  Constant/1 -> MATLAB Function/3(rotorPositions)
  Input/1 -> Thrust model/1(u), Torque model/1(u)
  Thrust model/1(thrustEachRotor) -> MATLAB Function/1(thrustEachRotor)
  Torque model/1(tauEachRotor) -> MATLAB Function/2(tauEachRotor)
  MATLAB Function/2(netM) -> M_rotors/1

== system PX4MultiCopterPerceptionAndControl/UAV Dynamics/Force and Moment Calculation/Ground Model/Friction Force ==
  V : Inport
  Fn : Inport  Port=2
  Product : Product
  Saturation : Saturate  UpperLimit=contact.translation.maxFriction  LowerLimit=-contact.translation.maxFriction
  Soft Coulomb Friction : Subsystem
  Unary Minus : UnaryMinus
  Friction : Outport
  wires:
  Fn/1 -> Product/2
  Soft Coulomb Friction/1(Out1) -> Product/1
  Product/1 -> Unary Minus/1
  V/1 -> Soft Coulomb Friction/1(In1)
  Unary Minus/1 -> Saturation/1
  Saturation/1 -> Friction/1

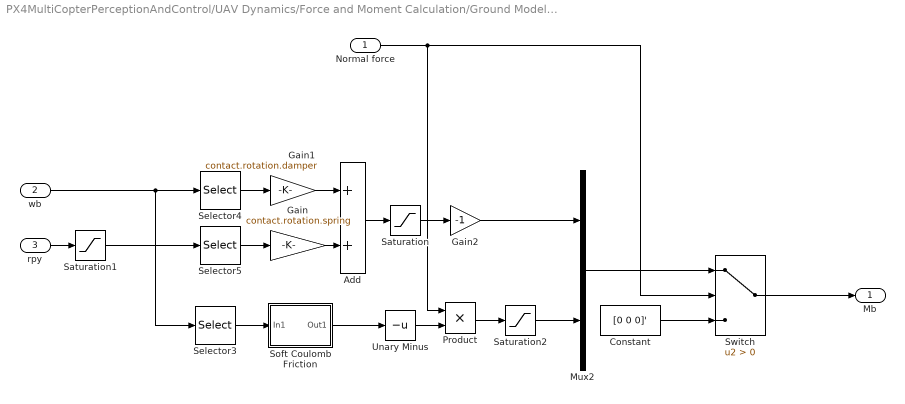
== system PX4MultiCopterPerceptionAndControl/UAV Dynamics/Force and Moment Calculation/Ground Model/Ground Moment Model ==
  Normal force : Inport
  wb : Inport  Port=2
  rpy : Inport  Port=3
  Add : Sum
  Constant : Constant  Value=[0 0 0]'
  Gain : Gain  Gain=contact.rotation.spring
  Gain1 : Gain  Gain=contact.rotation.damper
  Gain2 : Gain  Gain=-1
  Mux2 : Mux  Inputs=2
  Product : Product
  Saturation : Saturate  UpperLimit=control.rotation.maxMoment  LowerLimit=-control.rotation.maxMoment
  Saturation1 : Saturate  UpperLimit=20*pi/180  LowerLimit=-20*pi/180
  Saturation2 : Saturate  UpperLimit=control.rotation.maxMoment  LowerLimit=-control.rotation.maxMoment
  Selector3 : Selector  InputPortWidth=3  IndexOptions=Index vector (dialog)  Indices=[3]  OutputSizes=1
  Selector4 : Selector  InputPortWidth=3  IndexOptions=Index vector (dialog)  Indices=[1, 2]  OutputSizes=1
  Selector5 : Selector  InputPortWidth=3  IndexOptions=Index vector (dialog)  Indices=[1, 2]  OutputSizes=1
  Soft Coulomb Friction : Subsystem
  Switch : Switch  Criteria=u2 > Threshold  SaturateOnIntegerOverflow=off  InputSameDT=off
  Unary Minus : UnaryMinus
  Mb : Outport
  wires:
  Gain2/1 -> Mux2/1
  Add/1 -> Saturation/1
  Gain/1 -> Add/2
  Saturation/1 -> Gain2/1
  Selector4/1 -> Gain1/1
  Gain1/1 -> Add/1
  Constant/1 -> Switch/3
  Selector5/1 -> Gain/1
  Switch/1 -> Mb/1
  Mux2/1 -> Switch/1
  Normal force/1 -> Product/1, Switch/2
  rpy/1 -> Saturation1/1
  Saturation1/1 -> Selector5/1
  wb/1 -> Selector4/1, Selector3/1
  Selector3/1 -> Soft Coulomb Friction/1(In1)
  Soft Coulomb Friction/1(Out1) -> Unary Minus/1
  Unary Minus/1 -> Product/2
  Product/1 -> Saturation2/1
  Saturation2/1 -> Mux2/2

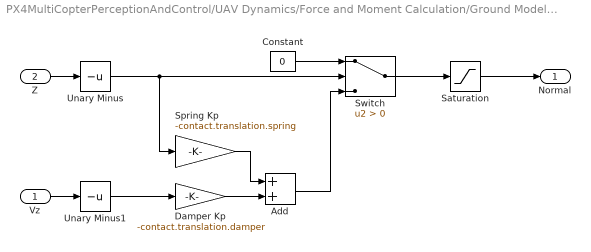
== system PX4MultiCopterPerceptionAndControl/UAV Dynamics/Force and Moment Calculation/Ground Model/Normal Force ==
  Vz : Inport
  Z : Inport  Port=2
  Add : Sum
  Constant : Constant  Value=0
  Damper Kp : Gain  Gain=-contact.translation.damper
  Saturation : Saturate  UpperLimit=contact.translation.maxNormal  LowerLimit=0
  Spring Kp : Gain  Gain=-contact.translation.spring
  Switch : Switch  Criteria=u2 > Threshold  SaturateOnIntegerOverflow=off  InputSameDT=off
  Unary Minus : UnaryMinus
  Unary Minus1 : UnaryMinus
  Normal : Outport
  wires:
  Constant/1 -> Switch/1
  Z/1 -> Unary Minus/1
  Switch/1 -> Saturation/1
  Damper Kp/1 -> Add/2
  Add/1 -> Switch/3
  Spring Kp/1 -> Add/1
  Vz/1 -> Unary Minus1/1
  Saturation/1 -> Normal/1
  Unary Minus/1 -> Spring Kp/1, Switch/2
  Unary Minus1/1 -> Damper Kp/1

== system PX4MultiCopterPerceptionAndControl/UAV Dynamics/Force and Moment Calculation/Rotor Model/Thrust model ==
  u : Inport
  Constant : Constant  Value=rotorThrustMax  SampleTime=SampleTime
  Constant1 : Constant  Value=rotorTimeConst  SampleTime=SampleTime
  Constant2 : Constant  Value=SampleTime  SampleTime=SampleTime
  MATLAB Function : MATLAB Function  TreatAsAtomicUnit=on
  Rate Transition1 : RateTransition
  Selector : Selector  InputPortWidth=8  IndexOptions=Index vector (dialog)  Indices=1:NoOfRotors  OutputSizes=1
  thrustEachRotor : Outport
  wires:
  u/1 -> Selector/1
  Selector/1 -> MATLAB Function/1(u)
  MATLAB Function/1(y) -> Rate Transition1/1
  Constant1/1 -> MATLAB Function/4(tau)
  Constant/1 -> MATLAB Function/3(K)
  Constant2/1 -> MATLAB Function/2(Ts)
  Rate Transition1/1 -> thrustEachRotor/1

== system PX4MultiCopterPerceptionAndControl/UAV Dynamics/Force and Moment Calculation/Rotor Model/Torque model ==
  u : Inport
  Constant : Constant  Value=rotorTorqueMax  SampleTime=SampleTime
  Constant1 : Constant  Value=rotorTimeConst  SampleTime=SampleTime
  Constant2 : Constant  Value=SampleTime  SampleTime=SampleTime
  MATLAB Function : MATLAB Function  TreatAsAtomicUnit=on
  Rate Transition : RateTransition
  Selector : Selector  InputPortWidth=8  IndexOptions=Index vector (dialog)  Indices=1:NoOfRotors  OutputSizes=1
  tauEachRotor : Outport
  wires:
  Constant1/1 -> MATLAB Function/4(tau)
  u/1 -> Selector/1
  MATLAB Function/1(y) -> Rate Transition/1
  Selector/1 -> MATLAB Function/1(u)
  Constant/1 -> MATLAB Function/3(K)
  Constant2/1 -> MATLAB Function/2(Ts)
  Rate Transition/1 -> tauEachRotor/1

== system PX4MultiCopterPerceptionAndControl/UAV Dynamics/Force and Moment Calculation/Ground Model/Friction Force/Soft Coulomb Friction ==
  note: Pennestrì, E., Rossi, V., Salvini, P. et al. Review and comparison of dry friction force models. Nonlinear Dyn 83, 1785–1801 (2016). https://doi.org/10.1007/s11071-015-2485-3
  In1 : Inport
  Tanh : Trigonometry  Operator=tanh
  friction coefficient : Gain  Gain=contact.translation.friction
  vd : Gain  Gain=1/contact.translation.vd
  Out1 : Outport
  wires:
  In1/1 -> vd/1
  vd/1 -> Tanh/1
  Tanh/1 -> friction coefficient/1
  friction coefficient/1 -> Out1/1

== system PX4MultiCopterPerceptionAndControl/UAV Dynamics/Force and Moment Calculation/Ground Model/Ground Moment Model/Soft Coulomb Friction ==
  note: Pennestrì, E., Rossi, V., Salvini, P. et al. Review and comparison of dry friction force models. Nonlinear Dyn 83, 1785–1801 (2016). https://doi.org/10.1007/s11071-015-2485-3
  In1 : Inport
  Tanh : Trigonometry  Operator=tanh
  friction coefficient : Gain  Gain=control.rotation.friction
  vd : Gain  Gain=1/control.rotation.vd
  Out1 : Outport
  wires:
  In1/1 -> vd/1
  vd/1 -> Tanh/1
  Tanh/1 -> friction coefficient/1
  friction coefficient/1 -> Out1/1

== matlab function PX4MultiCopterPerceptionAndControl/UAV Dynamics/Force and Moment Calculation/Aerodynamic drag/calcDragVector ==
  data: airVel input; dragVec output; dragCoeff input
function dragVec = fcn(airVel, dragCoeff)

dragVec = dragCoeff * norm(airVel) * airVel;

end

== matlab function PX4MultiCopterPerceptionAndControl/UAV Dynamics/Force and Moment Calculation/Rotor Model/MATLAB Function ==
  data: thrustEachRotor input; tauEachRotor input; rotorPositions input; netF output; netM output; rotorDir input
function [netF, netM] = getForceMoment(thrustEachRotor, tauEachRotor, rotorPositions, rotorDir)
%#codegen
Fx = 0;
Fy = 0;
Fz = -sum(thrustEachRotor);

netF = [Fx; Fy; Fz];

netM = [0; 0; 0]; %initialize
for i = 1:4
    rotPos = rotorPositions(:, i);
    Fi = [0, 0, -thrustEachRotor(i)]';
    netM = netM +  cross(rotPos, Fi);%contribution from thrusts of each propeller
    netM(3) = netM(3) - rotorDir(i)*tauEachRotor(i); %contribution from counter torque acting on propeller
end

end

== matlab function PX4MultiCopterPerceptionAndControl/UAV Dynamics/Force and Moment Calculation/Rotor Model/Thrust model/MATLAB Function ==
  data: u input; y output; Ts input; K input; tau input
function y = transferFcnVec(u, Ts, K, tau)
%#codegen
persistent y_prev
if isempty(y_prev)
    y_prev = zeros(size(u));
end

alpha = tau / (tau + Ts);
beta = K * Ts / (tau + Ts);

y = alpha .* y_prev + beta .* u;

y_prev = y;
end

== matlab function PX4MultiCopterPerceptionAndControl/UAV Dynamics/Force and Moment Calculation/Rotor Model/Torque model/MATLAB Function ==
  data: u input; y output; Ts input; K input; tau input
function y = transferFcnVec(u, Ts, K, tau)
%#codegen
persistent y_prev
if isempty(y_prev)
    y_prev = zeros(size(u));
end

alpha = tau / (tau + Ts);
beta = K * Ts / (tau + Ts);

y = alpha .* y_prev + beta .* u;

y_prev = y;
end

== matlab function PX4MultiCopterPerceptionAndControl/Visualization Subsystem/Subsystem1/MATLAB Function ==
  data: nedEuler input; ue4Euler output
function ue4Euler = convertNEDEulerToUE4(nedEuler)
    % Convert NED Euler angles to UE4 Euler angles with rotation order XZY
    % Assuming nedEuler is in degrees and in the order [pitch, roll, yaw]
    
    % Convert from NED (pitch, roll, yaw) to UE4 (roll, pitch, yaw)
    % Invert yaw for left-handed system
    ue4Euler = [nedEuler(3), nedEuler(2), nedEuler(1)];
	ue4Euler = reshape(ue4Euler, 1, 3);
end

== matlab function PX4MultiCopterPerceptionAndControl/Visualization Subsystem/Subsystem1/MATLAB Function1 ==
  data: nedCoords input; ue4Coords output
function ue4Coords  = convertNEDToUE4Translation(nedCoords)
	% Convert to UE4 coordinates
	ue4Coords = [nedCoords(1), nedCoords(2), -nedCoords(3)];
end

== matlab function PX4MultiCopterPerceptionAndControl/Visualization Subsystem/Subsystem1/MATLAB Function2 ==
  data: pos input; x_t output; y_t output; z_t output
function [x_t, y_t, z_t] = translate_point(pos)
    % Translation offsets
    dx = 0.5;
    dy = 1;
    dz = -0.046;
 
    % Apply translation
    x_t = pos(1) + dx;
    y_t = pos(2) + dy;
    z_t = pos(3) + dz;
end
